simulink model "clik_jacobian_inverse"  (R2023a)
settings: Solver=VariableStepAuto  StartTime=0.0  StopTime=5*24  RelTol=1e-3
undefined symbols (not defined in the file or in its folder): DiscIntNeverNeededParam, K, q0, Tc
settings Model: Creator=Valentina Giannotti  LastModifiedBy=salpi
settings OptimizationCC: ReuseModelBlockBuffer=off

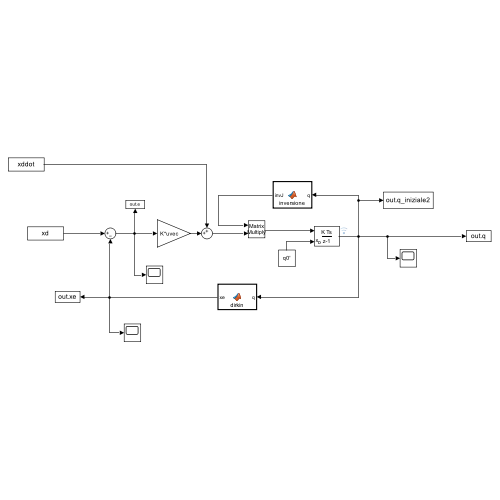
[thumbnail: Simulink's stored preview of the top-level diagram]
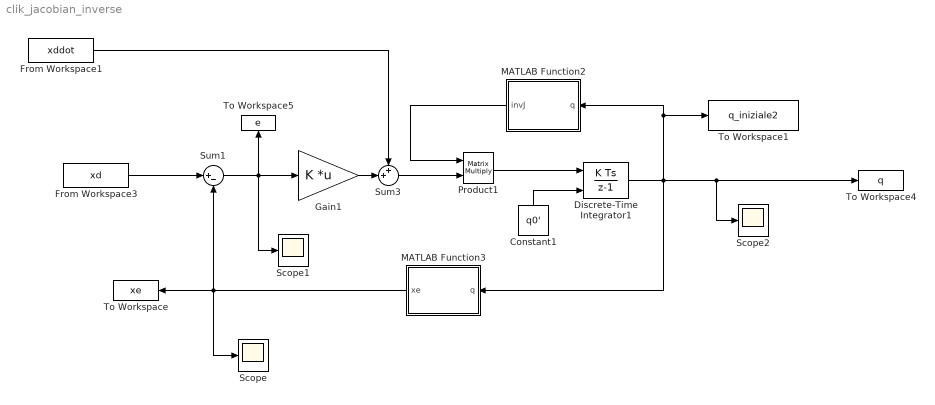
== system clik_jacobian_inverse ==
  Constant1 : Constant  Value=q0'  VectorParams1D=off
  Discrete-Time Integrator1 : DiscreteIntegrator  InitialConditionSource=external  InitialCondition=q0  SampleTime=Tc  ICPrevOutput=DiscIntNeverNeededParam  ICPrevScaledInput=DiscIntNeverNeededParam
  From Workspace1 : FromWorkspace  VariableName=xddot  SampleTime=Tc
  From Workspace3 : FromWorkspace  VariableName=xd  SampleTime=Tc
  Gain1 : Gain  Gain=K  Multiplication=Matrix(K*u) (u vector)
  MATLAB Function2 : MATLAB Function  TreatAsAtomicUnit=on
  MATLAB Function3 : MATLAB Function  TreatAsAtomicUnit=on
  Product1 : Product  Multiplication=Matrix(*)
  Scope : Scope
  Scope1 : Scope
  Scope2 : Scope
  Sum1 : Sum  Inputs=|+-
  Sum3 : Sum  Inputs=++|
  To Workspace : ToWorkspace  VariableName=xe  SaveFormat=Structure With Time  SampleTime=-1
  To Workspace1 : ToWorkspace  VariableName=q_iniziale2  SampleTime=-1
  To Workspace4 : ToWorkspace  VariableName=q  SaveFormat=Structure With Time  SampleTime=-1
  To Workspace5 : ToWorkspace  VariableName=e  SaveFormat=Structure With Time  SampleTime=-1
  wires:
  Sum1/1 -> Gain1/1, To Workspace5/1, Scope1/1
  Sum3/1 -> Product1/2
  MATLAB Function3/1(xe) -> Scope/1, To Workspace/1, Sum1/2
  Discrete-Time Integrator1/1 -> To Workspace1/1, MATLAB Function2/1(q), Scope2/1, To Workspace4/1, MATLAB Function3/1(q)
  MATLAB Function2/1(invJ) -> Product1/1
  Product1/1 -> Discrete-Time Integrator1/1
  Constant1/1 -> Discrete-Time Integrator1/2
  Gain1/1 -> Sum3/2
  From Workspace1/1 -> Sum3/1
  From Workspace3/1 -> Sum1/1

== matlab function clik_jacobian_inverse/MATLAB Function3 ==
  data: q input; xe output
function xe = dirkin(q)
% Pose in base coordinates, ordered as [x; y; z; phi].

a1 = 0.5;
a2 = 0.5;
d0 = 1;

xe = [a1*cos(q(1))+a2*cos(q(1)+q(2));
      a1*sin(q(1))+a2*sin(q(1)+q(2));
      d0+q(3);
      q(1)+q(2)+q(4)];

end

== matlab function clik_jacobian_inverse/MATLAB Function2 ==
  data: invJ output; q input
function invJ=inversione(q)
% Use the pseudoinverse of the full four-coordinate Jacobian.

a1 = 0.5;
a2 = 0.5;

J = [-a1*sin(q(1))-a2*sin(q(1)+q(2)) -a2*sin(q(1)+q(2)) 0 0;
      a1*cos(q(1))+a2*cos(q(1)+q(2))  a2*cos(q(1)+q(2)) 0 0;
                     0                         0        1 0;
                     1                         1        0 1];

invJ = pinv(J);

end
